simulink model "MotorTunerComparison"  (R2024b)
settings: Solver=FixedStepDiscrete  StartTime=0.0  StopTime=6  FixedStep=1e-4  RelTol=1e-3
InitFcn:
  | ccmp_init
undefined symbols (not defined in the file or in its folder): ccmpFuzzyKi, ccmpFuzzyKp, ccmpMethod, ccmpNN_b1, ccmpNN_b2, ccmpNN_W1, ccmpNN_W2, ccmpPlanKi, ccmpPlanKp, ccmpPlanTime, ccmpTD3_b1, ccmpTD3_b2, ccmpTD3_b3, ccmpTD3_W1, ccmpTD3_W2, ccmpTD3_W3, ccmpTD3ActionBias, ccmpTD3ActionScale, ccmpTD3Baseline, ccmpTD3Center, ccmpTD3InputMask, ccmpTD3KpLevels, ccmpTD3Scale
settings Model: DataDictionary=motor_comparison.sldd  Creator=lxy  LastModifiedBy=lxy
settings OptimizationCC: DefaultParameterBehavior=Inlined  UseDivisionForNetSlopeComputation=on  EnhancedBackFolding=on  PassReuseOutputArgsAs=Individual arguments  ZeroExternalMemoryAtStartup=off  ZeroInternalMemoryAtStartup=off  OptimizeBlockOrder=speed  DifferentSizesBufferReuse=on  OptimizationCustomize=off  EfficientTunableParamExpr=on
settings DebuggingCC: ParameterPrecisionLossMsg=none  ParameterTunabilityLossMsg=error
settings HardwareCC: ProdBitPerPointer=32  ProdBitPerSizeT=32  ProdBitPerPtrDiffT=32  ProdLargestAtomicInteger=Long  ProdLargestAtomicFloat=Double  ProdWordSize=32  ProdHWDeviceType=ARM Compatible->ARM Cortex-M
settings SFSimCC: MATLABDynamicMemAlloc=off
settings RTWCC: Description=Embedded Coder  SystemTargetFile=ert.tlc  TemplateMakefile=ert_default_tmf
settings CodeAppCC: ForceParamTrailComments=on  IgnoreCustomStorageClasses=off  OperatorAnnotations=on  SimulinkDataObjDesc=on  SFDataObjDesc=on  InsertBlockDesc=on
settings ERTTargetCC: TargetLangStandard=C99 (ISO)  GenerateSampleERTMain=on  ERTCustomFileTemplate=example_file_process.tlc

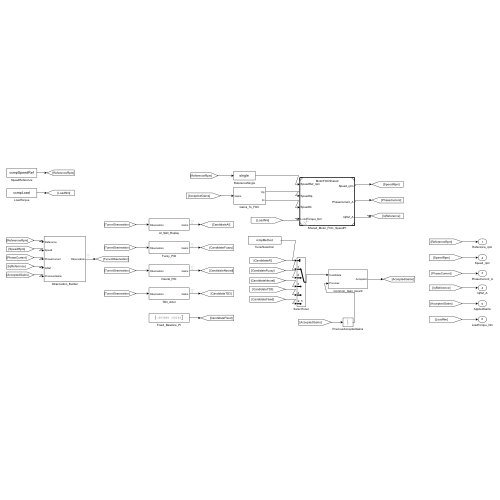
[thumbnail: Simulink's stored preview of the top-level diagram]
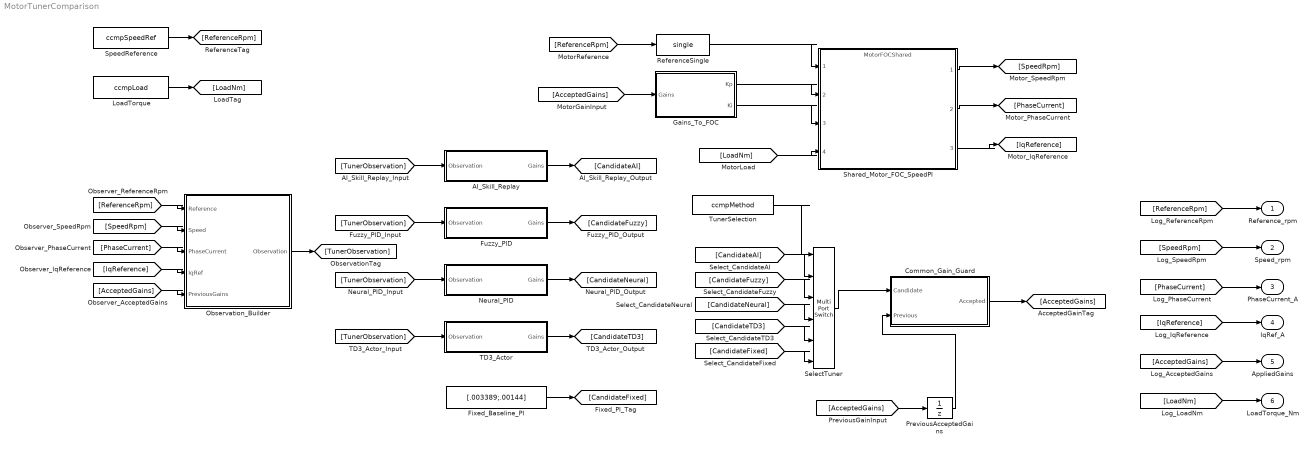
== system MotorTunerComparison ==
  AI_Skill_Replay : Subsystem
  Common_Gain_Guard : Subsystem
  Fixed_Baseline_PI : Constant  Value=[.003389;.00144]  SampleTime=0.1
  Fuzzy_PID : Subsystem
  Gains_To_FOC : Subsystem
  LoadTorque : FromWorkspace  VariableName=ccmpLoad  SampleTime=1e-4  Interpolate=off  OutputAfterFinalValue=Holding final value
  Neural_PID : Subsystem
  Observation_Builder : Subsystem
  PreviousAcceptedGains : UnitDelay  InitialCondition=[.003389;.00144]  SampleTime=0.1
  ReferenceSingle : DataTypeConversion  OutDataTypeStr=single
  SelectTuner : MultiPortSwitch  Inputs=5
  Shared_Motor_FOC_SpeedPI : ModelReference  ModelNameDialog=MotorFOCShared  SimulationMode=Normal  ModelReferenceVersion=7.2
  SpeedReference : FromWorkspace  VariableName=ccmpSpeedRef  SampleTime=1e-4  Interpolate=off  OutputAfterFinalValue=Holding final value
  TD3_Actor : Subsystem
  TunerSelection : Constant  Value=ccmpMethod  SampleTime=0.1
  Reference_rpm : Outport
  Speed_rpm : Outport  Port=2
  PhaseCurrent_A : Outport  Port=3
  IqRef_A : Outport  Port=4
  AppliedGains : Outport  Port=5
  LoadTorque_Nm : Outport  Port=6
  wires:
  [LoadNm] -> LoadTorque_Nm/1
  [AcceptedGains] -> AppliedGains/1
  [IqReference] -> IqRef_A/1
  [PhaseCurrent] -> PhaseCurrent_A/1
  [SpeedRpm] -> Speed_rpm/1
  [ReferenceRpm] -> Reference_rpm/1
  Shared_Motor_FOC_SpeedPI/3 -> [IqReference]
  Shared_Motor_FOC_SpeedPI/2 -> [PhaseCurrent]
  Shared_Motor_FOC_SpeedPI/1 -> [SpeedRpm]
  [LoadNm] -> Shared_Motor_FOC_SpeedPI/4
  ReferenceSingle/1 -> Shared_Motor_FOC_SpeedPI/1
  [ReferenceRpm] -> ReferenceSingle/1
  Gains_To_FOC/2(Ki) -> Shared_Motor_FOC_SpeedPI/3
  Gains_To_FOC/1(Kp) -> Shared_Motor_FOC_SpeedPI/2
  [AcceptedGains] -> Gains_To_FOC/1(Gains)
  Common_Gain_Guard/1(Accepted) -> [AcceptedGains]
  PreviousAcceptedGains/1 -> Common_Gain_Guard/2(Previous)
  [AcceptedGains] -> PreviousAcceptedGains/1
  SelectTuner/1 -> Common_Gain_Guard/1(Candidate)
  [CandidateFixed] -> SelectTuner/6
  [CandidateTD3] -> SelectTuner/5
  [CandidateNeural] -> SelectTuner/4
  [CandidateFuzzy] -> SelectTuner/3
  [CandidateAI] -> SelectTuner/2
  TunerSelection/1 -> SelectTuner/1
  Fixed_Baseline_PI/1 -> [CandidateFixed]
  TD3_Actor/1(Gains) -> [CandidateTD3]
  [TunerObservation] -> TD3_Actor/1(Observation)
  Neural_PID/1(Gains) -> [CandidateNeural]
  [TunerObservation] -> Neural_PID/1(Observation)
  Fuzzy_PID/1(Gains) -> [CandidateFuzzy]
  [TunerObservation] -> Fuzzy_PID/1(Observation)
  AI_Skill_Replay/1(Gains) -> [CandidateAI]
  [TunerObservation] -> AI_Skill_Replay/1(Observation)
  Observation_Builder/1(Observation) -> [TunerObservation]
  [AcceptedGains] -> Observation_Builder/5(PreviousGains)
  [IqReference] -> Observation_Builder/4(IqRef)
  [PhaseCurrent] -> Observation_Builder/3(PhaseCurrent)
  [SpeedRpm] -> Observation_Builder/2(Speed)
  [ReferenceRpm] -> Observation_Builder/1(Reference)
  LoadTorque/1 -> [LoadNm]
  SpeedReference/1 -> [ReferenceRpm]

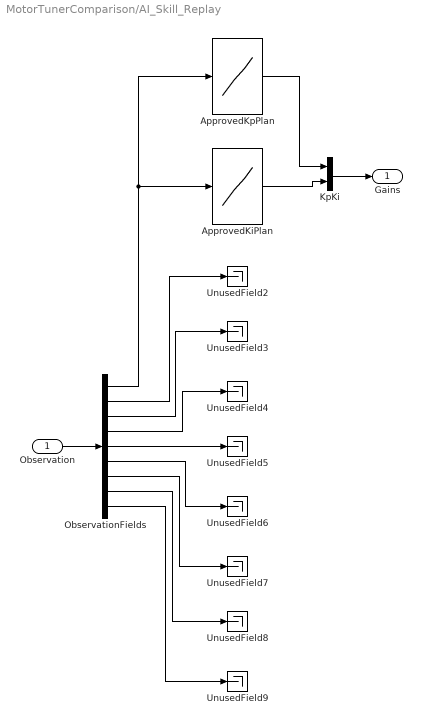
== system MotorTunerComparison/AI_Skill_Replay ==
  Observation : Inport
  ApprovedKiPlan : Lookup_n-D  NumberOfTableDimensions=1  BreakpointsForDimension1=ccmpPlanTime  Table=ccmpPlanKi  InterpMethod=Flat  ExtrapMethod=Clip
  ApprovedKpPlan : Lookup_n-D  NumberOfTableDimensions=1  BreakpointsForDimension1=ccmpPlanTime  Table=ccmpPlanKp  InterpMethod=Flat  ExtrapMethod=Clip
  KpKi : Mux  Inputs=2
  ObservationFields : Demux  Outputs=9
  UnusedField{2..9} (8 alike) : Terminator
  Gains : Outport
  wires:
  KpKi/1 -> Gains/1
  ApprovedKiPlan/1 -> KpKi/2
  ApprovedKpPlan/1 -> KpKi/1
  ObservationFields/1 -> ApprovedKpPlan/1, ApprovedKiPlan/1
  ObservationFields/9 -> UnusedField9/1
  ObservationFields/8 -> UnusedField8/1
  ObservationFields/7 -> UnusedField7/1
  ObservationFields/6 -> UnusedField6/1
  ObservationFields/5 -> UnusedField5/1
  ObservationFields/4 -> UnusedField4/1
  ObservationFields/3 -> UnusedField3/1
  ObservationFields/2 -> UnusedField2/1
  Observation/1 -> ObservationFields/1

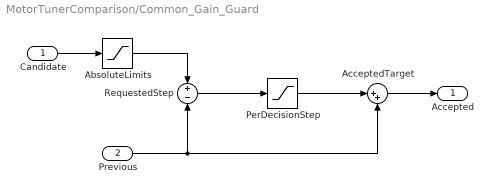
== system MotorTunerComparison/Common_Gain_Guard ==
  Candidate : Inport
  Previous : Inport  Port=2
  AbsoluteLimits : Saturate  UpperLimit=[.0054224;.00216]  LowerLimit=[.0013556;.00072]
  AcceptedTarget : Sum  Inputs=|++
  PerDecisionStep : Saturate  UpperLimit=[.00027112;.000144]  LowerLimit=[-.00027112;-.000144]
  RequestedStep : Sum  Inputs=+-
  Accepted : Outport
  wires:
  AcceptedTarget/1 -> Accepted/1
  PerDecisionStep/1 -> AcceptedTarget/1
  RequestedStep/1 -> PerDecisionStep/1
  Previous/1 -> RequestedStep/2, AcceptedTarget/2
  AbsoluteLimits/1 -> RequestedStep/1
  Candidate/1 -> AbsoluteLimits/1

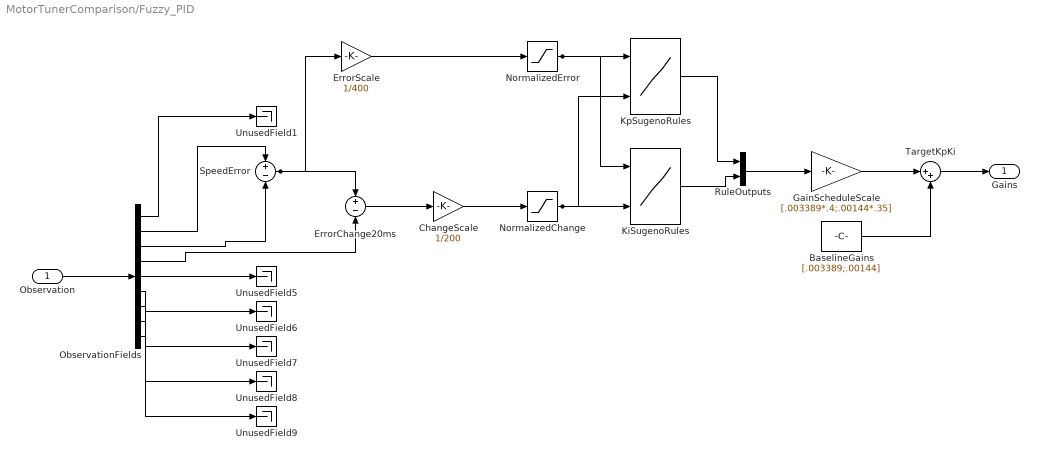
== system MotorTunerComparison/Fuzzy_PID ==
  Observation : Inport
  BaselineGains : Constant  Value=[.003389;.00144]  SampleTime=0.1
  ChangeScale : Gain  Gain=1/200
  ErrorChange20ms : Sum  Inputs=+-
  ErrorScale : Gain  Gain=1/400
  GainScheduleScale : Gain  Gain=[.003389*.4;.00144*.35]
  KiSugenoRules : Lookup_n-D  BreakpointsForDimension1=[-1 -.5 0 .5 1]  BreakpointsForDimension2=[-1 -.5 0 .5 1]  Table=ccmpFuzzyKi  ExtrapMethod=Clip
      settings: InputPortMap=u0,u1
  KpSugenoRules : Lookup_n-D  BreakpointsForDimension1=[-1 -.5 0 .5 1]  BreakpointsForDimension2=[-1 -.5 0 .5 1]  Table=ccmpFuzzyKp  ExtrapMethod=Clip
      settings: InputPortMap=u0,u1
  NormalizedChange : Saturate  UpperLimit=1  LowerLimit=-1
  NormalizedError : Saturate  UpperLimit=1  LowerLimit=-1
  ObservationFields : Demux  Outputs=9
  RuleOutputs : Mux  Inputs=2
  SpeedError : Sum  Inputs=+-
  TargetKpKi : Sum  Inputs=|++
  UnusedField{1,5..9} (6 alike) : Terminator
  Gains : Outport
  wires:
  NormalizedError/1 -> KiSugenoRules/1, KpSugenoRules/1
  ObservationFields/1 -> UnusedField1/1
  Observation/1 -> ObservationFields/1
  ObservationFields/2 -> SpeedError/1
  ObservationFields/3 -> SpeedError/2
  ObservationFields/4 -> ErrorChange20ms/2
  ObservationFields/5 -> UnusedField5/1
  ObservationFields/9 -> UnusedField9/1
  ObservationFields/8 -> UnusedField8/1
  ObservationFields/6 -> UnusedField6/1
  ObservationFields/7 -> UnusedField7/1
  RuleOutputs/1 -> GainScheduleScale/1
  SpeedError/1 -> ErrorChange20ms/1, ErrorScale/1
  ErrorChange20ms/1 -> ChangeScale/1
  ErrorScale/1 -> NormalizedError/1
  ChangeScale/1 -> NormalizedChange/1
  NormalizedChange/1 -> KiSugenoRules/2, KpSugenoRules/2
  KpSugenoRules/1 -> RuleOutputs/1
  KiSugenoRules/1 -> RuleOutputs/2
  GainScheduleScale/1 -> TargetKpKi/1
  BaselineGains/1 -> TargetKpKi/2
  TargetKpKi/1 -> Gains/1

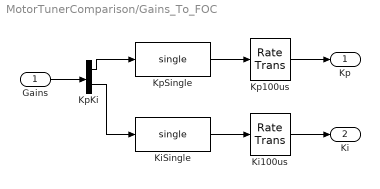
== system MotorTunerComparison/Gains_To_FOC ==
  Gains : Inport
  Ki100us : RateTransition  OutPortSampleTime=1e-4
  KiSingle : DataTypeConversion  OutDataTypeStr=single
  Kp100us : RateTransition  OutPortSampleTime=1e-4
  KpKi : Demux  Outputs=2
  KpSingle : DataTypeConversion  OutDataTypeStr=single
  Kp : Outport
  Ki : Outport  Port=2
  wires:
  Gains/1 -> KpKi/1
  Kp100us/1 -> Kp/1
  KpKi/1 -> KpSingle/1
  KpSingle/1 -> Kp100us/1
  KpKi/2 -> KiSingle/1
  KiSingle/1 -> Ki100us/1
  Ki100us/1 -> Ki/1

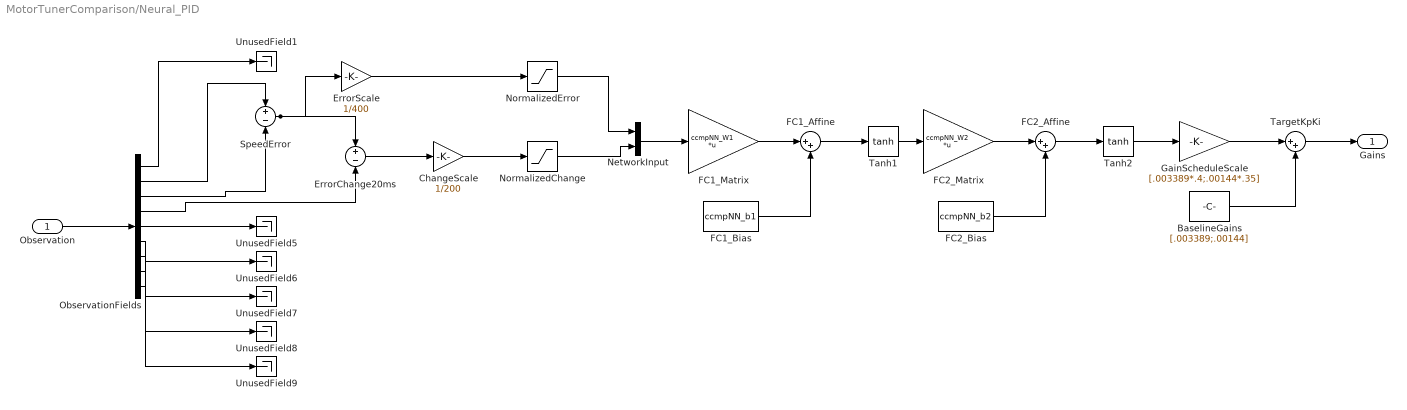
== system MotorTunerComparison/Neural_PID ==
  Observation : Inport
  BaselineGains : Constant  Value=[.003389;.00144]  SampleTime=0.1
  ChangeScale : Gain  Gain=1/200
  ErrorChange20ms : Sum  Inputs=+-
  ErrorScale : Gain  Gain=1/400
  FC1_Affine : Sum  Inputs=|++
  FC1_Bias : Constant  Value=ccmpNN_b1  SampleTime=0.1
  FC1_Matrix : Gain  Gain=ccmpNN_W1  Multiplication=Matrix(K*u)
  FC2_Affine : Sum  Inputs=|++
  FC2_Bias : Constant  Value=ccmpNN_b2  SampleTime=0.1
  FC2_Matrix : Gain  Gain=ccmpNN_W2  Multiplication=Matrix(K*u)
  GainScheduleScale : Gain  Gain=[.003389*.4;.00144*.35]
  NetworkInput : Mux  Inputs=2
  NormalizedChange : Saturate  UpperLimit=1  LowerLimit=-1
  NormalizedError : Saturate  UpperLimit=1  LowerLimit=-1
  ObservationFields : Demux  Outputs=9
  SpeedError : Sum  Inputs=+-
  Tanh1 : Trigonometry  Operator=tanh
  Tanh2 : Trigonometry  Operator=tanh
  TargetKpKi : Sum  Inputs=|++
  UnusedField{1,5..9} (6 alike) : Terminator
  Gains : Outport
  wires:
  Observation/1 -> ObservationFields/1
  ObservationFields/1 -> UnusedField1/1
  ObservationFields/2 -> SpeedError/1
  ObservationFields/3 -> SpeedError/2
  ObservationFields/4 -> ErrorChange20ms/2
  ObservationFields/8 -> UnusedField8/1
  ObservationFields/5 -> UnusedField5/1
  ObservationFields/6 -> UnusedField6/1
  ObservationFields/7 -> UnusedField7/1
  ObservationFields/9 -> UnusedField9/1
  Tanh1/1 -> FC2_Matrix/1
  SpeedError/1 -> ErrorChange20ms/1, ErrorScale/1
  ErrorScale/1 -> NormalizedError/1
  ErrorChange20ms/1 -> ChangeScale/1
  BaselineGains/1 -> TargetKpKi/2
  ChangeScale/1 -> NormalizedChange/1
  NormalizedError/1 -> NetworkInput/1
  NetworkInput/1 -> FC1_Matrix/1
  NormalizedChange/1 -> NetworkInput/2
  FC1_Bias/1 -> FC1_Affine/2
  FC1_Matrix/1 -> FC1_Affine/1
  FC1_Affine/1 -> Tanh1/1
  GainScheduleScale/1 -> TargetKpKi/1
  FC2_Matrix/1 -> FC2_Affine/1
  FC2_Bias/1 -> FC2_Affine/2
  FC2_Affine/1 -> Tanh2/1
  Tanh2/1 -> GainScheduleScale/1
  TargetKpKi/1 -> Gains/1

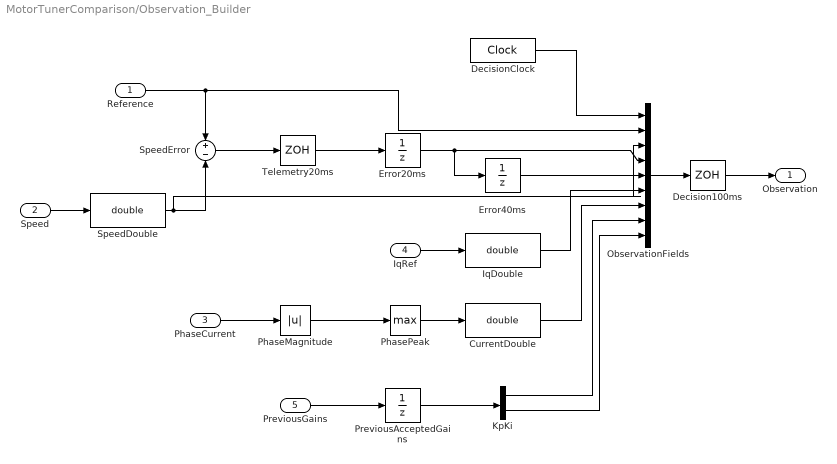
== system MotorTunerComparison/Observation_Builder ==
  Reference : Inport
  Speed : Inport  Port=2
  PhaseCurrent : Inport  Port=3
  IqRef : Inport  Port=4
  PreviousGains : Inport  Port=5
  CurrentDouble : DataTypeConversion  OutDataTypeStr=double
  Decision100ms : ZeroOrderHold  SampleTime=0.1
  DecisionClock : DigitalClock  SampleTime=0.1
  Error20ms : UnitDelay  SampleTime=0.02
  Error40ms : UnitDelay  SampleTime=0.02
  IqDouble : DataTypeConversion  OutDataTypeStr=double
  KpKi : Demux  Outputs=2
  ObservationFields : Mux  Inputs=9
  PhaseMagnitude : Abs
  PhasePeak : MinMax  Function=max
  PreviousAcceptedGains : UnitDelay  InitialCondition=[.003389;.00144]  SampleTime=0.1
  SpeedDouble : DataTypeConversion  OutDataTypeStr=double
  SpeedError : Sum  Inputs=+-
  Telemetry20ms : ZeroOrderHold  SampleTime=0.02
  Observation : Outport
  wires:
  Decision100ms/1 -> Observation/1
  ObservationFields/1 -> Decision100ms/1
  KpKi/2 -> ObservationFields/9
  KpKi/1 -> ObservationFields/8
  CurrentDouble/1 -> ObservationFields/7
  IqDouble/1 -> ObservationFields/6
  Error40ms/1 -> ObservationFields/5
  DecisionClock/1 -> ObservationFields/1
  PreviousAcceptedGains/1 -> KpKi/1
  PreviousGains/1 -> PreviousAcceptedGains/1
  Error20ms/1 -> Error40ms/1, ObservationFields/4
  Telemetry20ms/1 -> Error20ms/1
  SpeedError/1 -> Telemetry20ms/1
  SpeedDouble/1 -> SpeedError/2, ObservationFields/3
  Reference/1 -> SpeedError/1, ObservationFields/2
  PhasePeak/1 -> CurrentDouble/1
  PhaseMagnitude/1 -> PhasePeak/1
  PhaseCurrent/1 -> PhaseMagnitude/1
  IqRef/1 -> IqDouble/1
  Speed/1 -> SpeedDouble/1

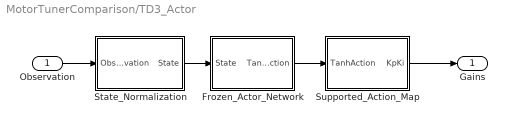
== system MotorTunerComparison/TD3_Actor ==
  Observation : Inport
  Frozen_Actor_Network : Subsystem
  State_Normalization : Subsystem
  Supported_Action_Map : Subsystem
  Gains : Outport
  wires:
  Supported_Action_Map/1(KpKi) -> Gains/1
  Frozen_Actor_Network/1(TanhAction) -> Supported_Action_Map/1(TanhAction)
  State_Normalization/1(State) -> Frozen_Actor_Network/1(State)
  Observation/1 -> State_Normalization/1(Observation)

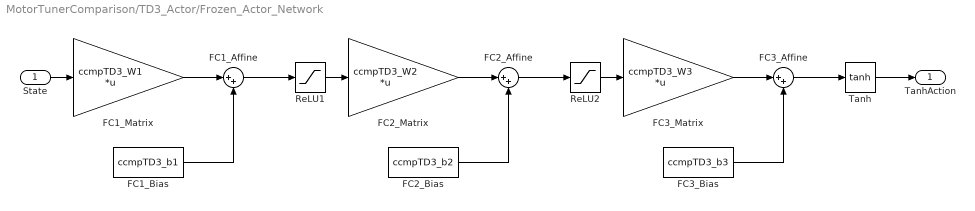
== system MotorTunerComparison/TD3_Actor/Frozen_Actor_Network ==
  State : Inport
  FC1_Affine : Sum  Inputs=|++
  FC1_Bias : Constant  Value=ccmpTD3_b1  SampleTime=0.1
  FC1_Matrix : Gain  Gain=ccmpTD3_W1  Multiplication=Matrix(K*u)
  FC2_Affine : Sum  Inputs=|++
  FC2_Bias : Constant  Value=ccmpTD3_b2  SampleTime=0.1
  FC2_Matrix : Gain  Gain=ccmpTD3_W2  Multiplication=Matrix(K*u)
  FC3_Affine : Sum  Inputs=|++
  FC3_Bias : Constant  Value=ccmpTD3_b3  SampleTime=0.1
  FC3_Matrix : Gain  Gain=ccmpTD3_W3  Multiplication=Matrix(K*u)
  ReLU1 : Saturate  UpperLimit=inf  LowerLimit=0
  ReLU2 : Saturate  UpperLimit=inf  LowerLimit=0
  Tanh : Trigonometry  Operator=tanh
  TanhAction : Outport
  wires:
  ReLU2/1 -> FC3_Matrix/1
  ReLU1/1 -> FC2_Matrix/1
  State/1 -> FC1_Matrix/1
  FC1_Matrix/1 -> FC1_Affine/1
  FC1_Bias/1 -> FC1_Affine/2
  FC1_Affine/1 -> ReLU1/1
  FC2_Matrix/1 -> FC2_Affine/1
  FC2_Bias/1 -> FC2_Affine/2
  FC2_Affine/1 -> ReLU2/1
  FC3_Matrix/1 -> FC3_Affine/1
  FC3_Affine/1 -> Tanh/1
  FC3_Bias/1 -> FC3_Affine/2
  Tanh/1 -> TanhAction/1

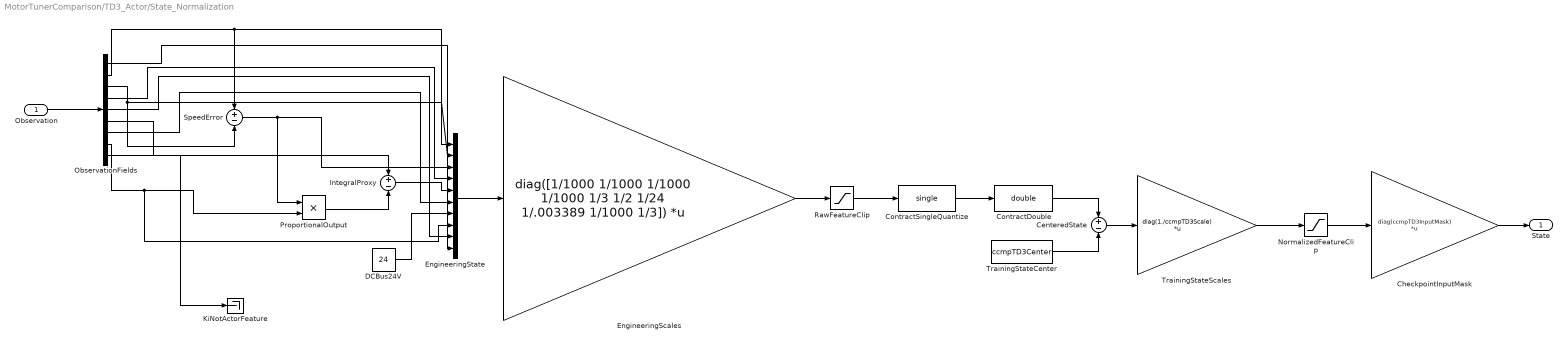
== system MotorTunerComparison/TD3_Actor/State_Normalization ==
  Observation : Inport
  CenteredState : Sum  Inputs=+-
  CheckpointInputMask : Gain  Gain=diag(ccmpTD3InputMask)  Multiplication=Matrix(K*u)
  ContractDouble : DataTypeConversion  OutDataTypeStr=double
  ContractSingleQuantize : DataTypeConversion  OutDataTypeStr=single
  DCBus24V : Constant  Value=24  SampleTime=0.1
  EngineeringScales : Gain  Gain=diag([1/1000 1/1000 1/1000 1/1000 1/3 1/2 1/24 1/.003389 1/1000 1/3])  Multiplication=Matrix(K*u)
  EngineeringState : Mux  Inputs=10
  IntegralProxy : Sum  Inputs=+-
  KiNotActorFeature : Terminator
  NormalizedFeatureClip : Saturate  UpperLimit=5  LowerLimit=-5
  ObservationFields : Demux  Outputs=9
  ProportionalOutput : Product
  RawFeatureClip : Saturate  UpperLimit=5  LowerLimit=-5
  SpeedError : Sum  Inputs=+-
  TrainingStateCenter : Constant  Value=ccmpTD3Center  SampleTime=0.1
  TrainingStateScales : Gain  Gain=diag(1./ccmpTD3Scale)  Multiplication=Matrix(K*u)
  State : Outport
  wires:
  SpeedError/1 -> ProportionalOutput/1, EngineeringState/3
  Observation/1 -> ObservationFields/1
  ObservationFields/1 -> EngineeringState/10
  ObservationFields/2 -> EngineeringState/1, SpeedError/1
  ObservationFields/3 -> SpeedError/2, EngineeringState/2
  ObservationFields/4 -> EngineeringState/4
  ObservationFields/8 -> EngineeringState/8, ProportionalOutput/2
  ObservationFields/5 -> EngineeringState/9
  ObservationFields/6 -> IntegralProxy/1
  ObservationFields/7 -> EngineeringState/6
  ObservationFields/9 -> KiNotActorFeature/1
  RawFeatureClip/1 -> ContractSingleQuantize/1
  IntegralProxy/1 -> EngineeringState/5
  ProportionalOutput/1 -> IntegralProxy/2
  DCBus24V/1 -> EngineeringState/7
  EngineeringState/1 -> EngineeringScales/1
  EngineeringScales/1 -> RawFeatureClip/1
  ContractDouble/1 -> CenteredState/1
  ContractSingleQuantize/1 -> ContractDouble/1
  TrainingStateCenter/1 -> CenteredState/2
  CenteredState/1 -> TrainingStateScales/1
  TrainingStateScales/1 -> NormalizedFeatureClip/1
  NormalizedFeatureClip/1 -> CheckpointInputMask/1
  CheckpointInputMask/1 -> State/1

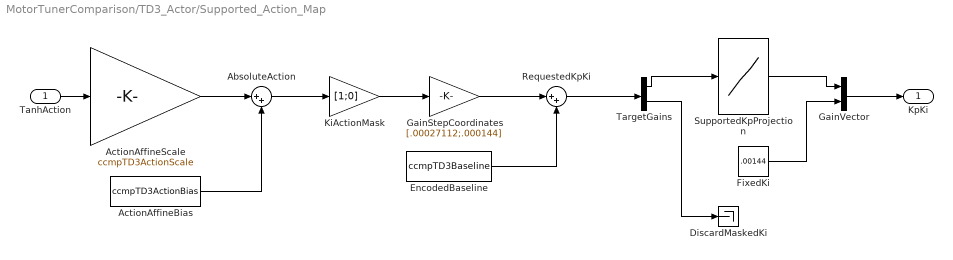
== system MotorTunerComparison/TD3_Actor/Supported_Action_Map ==
  TanhAction : Inport
  AbsoluteAction : Sum  Inputs=|++
  ActionAffineBias : Constant  Value=ccmpTD3ActionBias  SampleTime=0.1
  ActionAffineScale : Gain  Gain=ccmpTD3ActionScale
  DiscardMaskedKi : Terminator
  EncodedBaseline : Constant  Value=ccmpTD3Baseline  SampleTime=0.1
  FixedKi : Constant  Value=.00144  SampleTime=0.1
  GainStepCoordinates : Gain  Gain=[.00027112;.000144]
  GainVector : Mux  Inputs=2
  KiActionMask : Gain  Gain=[1;0]
  RequestedKpKi : Sum  Inputs=|++
  SupportedKpProjection : Lookup_n-D  NumberOfTableDimensions=1  BreakpointsForDimension1=ccmpTD3KpLevels  Table=ccmpTD3KpLevels  InterpMethod=Nearest  ExtrapMethod=Clip
  TargetGains : Demux  Outputs=2
  KpKi : Outport
  wires:
  RequestedKpKi/1 -> TargetGains/1
  TanhAction/1 -> ActionAffineScale/1
  ActionAffineScale/1 -> AbsoluteAction/1
  ActionAffineBias/1 -> AbsoluteAction/2
  AbsoluteAction/1 -> KiActionMask/1
  KiActionMask/1 -> GainStepCoordinates/1
  GainStepCoordinates/1 -> RequestedKpKi/1
  FixedKi/1 -> GainVector/2
  EncodedBaseline/1 -> RequestedKpKi/2
  SupportedKpProjection/1 -> GainVector/1
  TargetGains/2 -> DiscardMaskedKi/1
  TargetGains/1 -> SupportedKpProjection/1
  GainVector/1 -> KpKi/1
